simulink model "Collision_avoidance"  (R2025a)
settings: Solver=VariableStepAuto  StartTime=0.0  StopTime=30  RelTol=1e-3
InitFcn:
  | %% Simulation parameters and waypoint trajectory
  | % Initial drone positions.
  | init_0=[0;0;0];
  | d_s=4;
  | init_1=init_0+d_s*[-1.1;0.1;0];
  | init_2=init_0+d_s*[0.3;-1.5;0];
  | init_3=init_0+d_s*[0.2;1.8;0];
  | init_4=init_0+d_s*[1.6;0.4;0];
  | 
  | Threshold = 1000*ones(45,1);
  | for i=1:9:37
  |     Threshold(i:i+2)=10;
  | end
  | gain_2=1;
  | 
  | % Desired formation offsets.
  | init_f_0=[0;0;0];
  | d_f=1;
  | init_f_1=init_0+d_f*[0;-1;0];
  | init_f_2=init_0+d_f*[-1;0;0];
  | init_f_3=init_0+d_f*[1;0;0];
  | init_f_4=init_0+d_f*[0;1;0];
  | 
  | % Quadrotor mass and inertia.
  | mass = 1.2;
  | Ib   = diag([1.2416 1.2416 2*1.2416]);
  | 
  | % Time grid and waypoint trajectory.
  | Ts        = 0.001;
  | ttot      = 20;
  | tdead     = 10;
  | totalTime = ttot + tdead;
  | Nsamples  = 3000;
  | t_sample  = linspace(0, totalTime, Nsamples);
  | t=t_sample;
  | waypoints = [ ...
  |              0  0 0 0;
  |              0  0 0 0;
  |              0  0 0 0;
  |              0 0 0 0];
  | 
  | M    = size(waypoints,1);
  | t_wp = linspace(0, ttot, M);
  | 
  | p_d      = zeros(4, Nsamples);
  | dot_p_d  = zeros(4, Nsamples);
  | ddot_p_d = zeros(4, Nsamples);
  | 
  | idx_traj = t_sample <= ttot;
  | t_active = t_sample(idx_traj);
  | 
  | % Build position and yaw splines with zero endpoint velocities.
  | for dim = 1:4
  |     pp  = spline(t_wp, [0, waypoints(:,dim)&apos;, 0]);
  |     pp1 = fnder(pp,1);
  |     pp2 = fnder(pp,2);
  | 
  |     p_d(dim,    idx_traj) = ppval(pp,  t_active);
  |     dot_p_d(dim,idx_traj) = ppval(pp1, t_active);
  |     ddot_p_d(dim,idx_traj)= ppval(pp2, t_active);
  | end
  | 
  | % Hold the final waypoint after the maneuver.
  | last_wp_idx = M;
  | p_d(:, ~idx_traj)      = repmat(waypoints(last_wp_idx,:)&apos;, 1, sum(~idx_traj));
  | dot_p_d(:, ~idx_traj)  = 0;
  | ddot_p_d(:, ~idx_traj) = 0;
  | 
  | % Reference signals used by the Simulink blocks.
  | csi_d      = p_d(1:3,:);
  | psi_d      = p_d(4,:);
  | 
  | dot_csi_d  = dot_p_d(1:3,:);
  | ddot_csi_d = ddot_p_d(1:3,:);
  | dot_psi_d  = dot_p_d(4,:);
  | ddot_psi_d = ddot_p_d(4,:);
  | 
  | pos_0     = waypoints(1,1:3);
  | lin_vel_0 = [0 0 0];
  | w_bb_0    = [0 0 0];
undefined symbols (not defined in the file): A_diacenza, K
libraries: robotcorelib x5, uavutilslib x1
(part 1 of 2)
settings Model: Creator=fabioruggiero  LastModifiedBy=Giammo
settings ModelReferenceCC: EnableRefExpFcnMdlSchedulingChecks=on
settings RTWCC: GPUComputeCapability=3.5

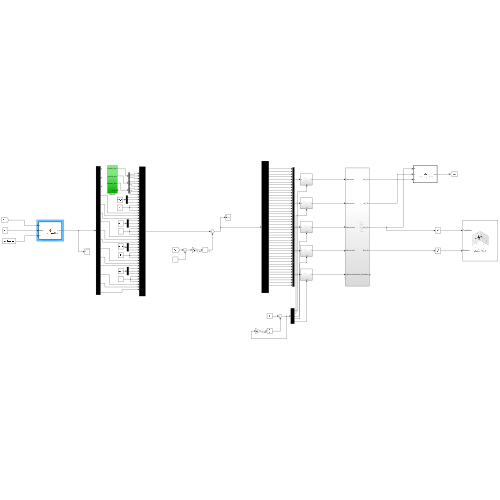
[thumbnail: Simulink's stored preview of the top-level diagram]
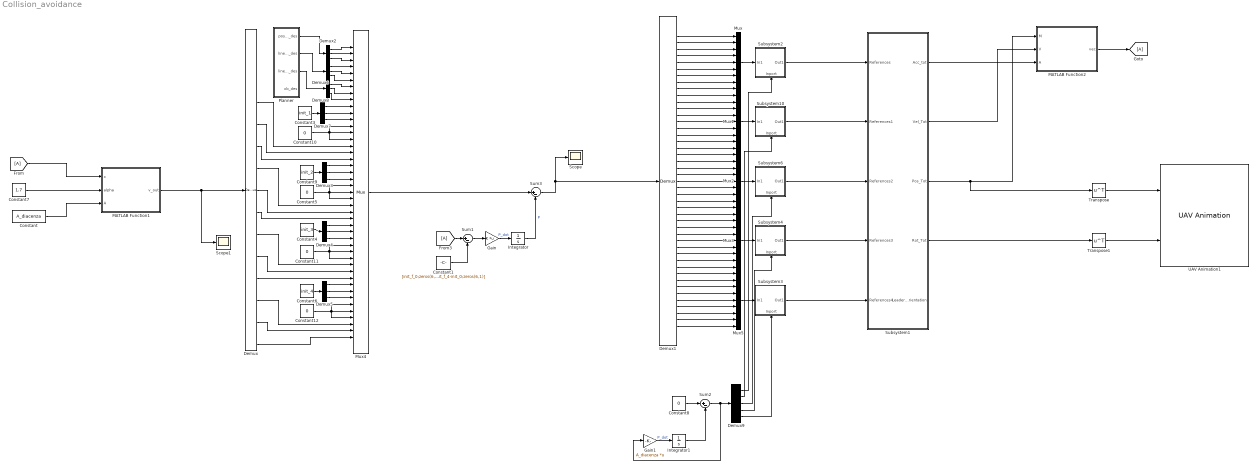
== system Collision_avoidance ==
  Constant : Constant  Value=A_diacenza
  Constant1 : Constant  Value=[init_f_0;zeros(6,1);init_f_1-init_0;zeros(6,1);init_f_2-init_0;zeros(6,1);init_f_3-init_0;zeros(6,1);init_f_4-init_0;zeros(6,1)]
  Constant{5,8,10..12} (5 alike) : Constant  Value=0
  Constant3 : Constant  Value=init_1
  Constant4 : Constant  Value=init_3
  Constant6 : Constant  Value=init_4
  Constant7 : Constant  Value=1.7
  Constant9 : Constant  Value=init_2
  Demux : Demux  Outputs=15
  Demux1 : Demux  Outputs=45
  Demux{2..8} (7 alike) : Demux  Outputs=3
  Demux9 : Demux  Outputs=5
  From : From
  From3 : From
  Gain : Gain  Gain=K  Multiplication=Matrix(K*u)
  Gain1 : Gain  Gain=A_diacenza  Multiplication=Matrix(K*u)
  Goto : Goto
  Integrator : Integrator
  Integrator1 : Integrator
  MATLAB Function1 : MATLAB Function  TreatAsAtomicUnit=on
  MATLAB Function2 : MATLAB Function  TreatAsAtomicUnit=on
  Mux{,1..3,5} (5 alike) : Mux  Inputs=9
  Mux4 : Mux  Inputs=45
  Planner : Subsystem
  Scope : Scope
      settings: ActiveDisplayYMinimum=-34.636381337350009  ActiveDisplayYMaximum=35.165535436651609  DataLoggingVariableName=ScopeData6
  Scope1 : Scope
      settings: ActiveDisplayYMinimum=-76.54569903346453  ActiveDisplayYMaximum=69.602196273492  DataLoggingVariableName=ScopeData7
  Subsystem1 : Subsystem
  Subsystem10 : Subsystem
      settings: PortSchema="{\"entries\":[{\"content\":{\"sides\":[{\"content\":{\"connectorIds\":[\"In1\"]},\"type\":\"ConnectorPlacement.EquallySpacedRectSide\",\"uuid\":\"6e5d8b99-8054-458f-abbe-7e3d6126420c\"},{\"content\":{\"connectorIds\":[\"Out1\"],\"side\":\"RIGHT\"},\"type\":\"ConnectorPlacement.EquallySpacedRectSide\",\"uuid\":\"d8af8c34-1227-4a19-bfdc-b42d943ed13c\"},{\"content\":{\"side\":\"TOP\"},\"type\":\"ConnectorPlacement.EquallySpacedRectSide\",\"uuid\":\"9c10b933-2873-4349-b535-f2af5c16ec70\"},{\"content\":{\"connectorIds\":[\"In2\"],\"side\":\"BOTTOM\"},\"type\":\"ConnectorPlacement.EquallySpacedRectSide\",\"uuid\":\"05be8d01-ed26-4f96-bcb1-0e501cb43bcc\"}]},\"type\":\"ConnectorPlacement.EquallySpacedConnector\",\"uuid\":\"f87e25de-488b-44c6-b2e5-9d22d609821c\"}],\"packageUris\":[\"http://schema.mathworks.com/mf0/Connector/R2020b\"],\"version\":\"1.0\"}"
  Subsystem2 : Subsystem
      settings: PortSchema="{\"entries\":[{\"content\":{\"sides\":[{\"content\":{\"connectorIds\":[\"In1\"]},\"type\":\"ConnectorPlacement.EquallySpacedRectSide\",\"uuid\":\"6e5d8b99-8054-458f-abbe-7e3d6126420c\"},{\"content\":{\"connectorIds\":[\"Out1\"],\"side\":\"RIGHT\"},\"type\":\"ConnectorPlacement.EquallySpacedRectSide\",\"uuid\":\"d8af8c34-1227-4a19-bfdc-b42d943ed13c\"},{\"content\":{\"side\":\"TOP\"},\"type\":\"ConnectorPlacement.EquallySpacedRectSide\",\"uuid\":\"9c10b933-2873-4349-b535-f2af5c16ec70\"},{\"content\":{\"connectorIds\":[\"In2\"],\"side\":\"BOTTOM\"},\"type\":\"ConnectorPlacement.EquallySpacedRectSide\",\"uuid\":\"05be8d01-ed26-4f96-bcb1-0e501cb43bcc\"}]},\"type\":\"ConnectorPlacement.EquallySpacedConnector\",\"uuid\":\"f87e25de-488b-44c6-b2e5-9d22d609821c\"}],\"packageUris\":[\"http://schema.mathworks.com/mf0/Connector/R2020b\"],\"version\":\"1.0\"}"
  Subsystem3 : Subsystem
      settings: PortSchema="{\"entries\":[{\"content\":{\"sides\":[{\"content\":{\"connectorIds\":[\"In1\"]},\"type\":\"ConnectorPlacement.EquallySpacedRectSide\",\"uuid\":\"6e5d8b99-8054-458f-abbe-7e3d6126420c\"},{\"content\":{\"connectorIds\":[\"Out1\"],\"side\":\"RIGHT\"},\"type\":\"ConnectorPlacement.EquallySpacedRectSide\",\"uuid\":\"d8af8c34-1227-4a19-bfdc-b42d943ed13c\"},{\"content\":{\"side\":\"TOP\"},\"type\":\"ConnectorPlacement.EquallySpacedRectSide\",\"uuid\":\"9c10b933-2873-4349-b535-f2af5c16ec70\"},{\"content\":{\"connectorIds\":[\"In2\"],\"side\":\"BOTTOM\"},\"type\":\"ConnectorPlacement.EquallySpacedRectSide\",\"uuid\":\"05be8d01-ed26-4f96-bcb1-0e501cb43bcc\"}]},\"type\":\"ConnectorPlacement.EquallySpacedConnector\",\"uuid\":\"f87e25de-488b-44c6-b2e5-9d22d609821c\"}],\"packageUris\":[\"http://schema.mathworks.com/mf0/Connector/R2020b\"],\"version\":\"1.0\"}"
  Subsystem4 : Subsystem
      settings: PortSchema="{\"entries\":[{\"content\":{\"sides\":[{\"content\":{\"connectorIds\":[\"In1\"]},\"type\":\"ConnectorPlacement.EquallySpacedRectSide\",\"uuid\":\"6e5d8b99-8054-458f-abbe-7e3d6126420c\"},{\"content\":{\"connectorIds\":[\"Out1\"],\"side\":\"RIGHT\"},\"type\":\"ConnectorPlacement.EquallySpacedRectSide\",\"uuid\":\"d8af8c34-1227-4a19-bfdc-b42d943ed13c\"},{\"content\":{\"side\":\"TOP\"},\"type\":\"ConnectorPlacement.EquallySpacedRectSide\",\"uuid\":\"9c10b933-2873-4349-b535-f2af5c16ec70\"},{\"content\":{\"connectorIds\":[\"In2\"],\"side\":\"BOTTOM\"},\"type\":\"ConnectorPlacement.EquallySpacedRectSide\",\"uuid\":\"05be8d01-ed26-4f96-bcb1-0e501cb43bcc\"}]},\"type\":\"ConnectorPlacement.EquallySpacedConnector\",\"uuid\":\"f87e25de-488b-44c6-b2e5-9d22d609821c\"}],\"packageUris\":[\"http://schema.mathworks.com/mf0/Connector/R2020b\"],\"version\":\"1.0\"}"
  Subsystem6 : Subsystem
      settings: PortSchema="{\"entries\":[{\"content\":{\"sides\":[{\"content\":{\"connectorIds\":[\"In1\"]},\"type\":\"ConnectorPlacement.EquallySpacedRectSide\",\"uuid\":\"6e5d8b99-8054-458f-abbe-7e3d6126420c\"},{\"content\":{\"connectorIds\":[\"Out1\"],\"side\":\"RIGHT\"},\"type\":\"ConnectorPlacement.EquallySpacedRectSide\",\"uuid\":\"d8af8c34-1227-4a19-bfdc-b42d943ed13c\"},{\"content\":{\"side\":\"TOP\"},\"type\":\"ConnectorPlacement.EquallySpacedRectSide\",\"uuid\":\"9c10b933-2873-4349-b535-f2af5c16ec70\"},{\"content\":{\"connectorIds\":[\"In2\"],\"side\":\"BOTTOM\"},\"type\":\"ConnectorPlacement.EquallySpacedRectSide\",\"uuid\":\"05be8d01-ed26-4f96-bcb1-0e501cb43bcc\"}]},\"type\":\"ConnectorPlacement.EquallySpacedConnector\",\"uuid\":\"f87e25de-488b-44c6-b2e5-9d22d609821c\"}],\"packageUris\":[\"http://schema.mathworks.com/mf0/Connector/R2020b\"],\"version\":\"1.0\"}"
  Sum1 : Sum  Inputs=|+-
  Sum2 : Sum  Inputs=|+-
  Sum3 : Sum  Inputs=|+-
  Transpose : Math  Operator=transpose
  Transpose1 : Math  Operator=transpose
  UAV Animation1 : uavutilslib/UAV Animation  NumUAV=5  DynamicUAVConfig=off  UAVType=Multirotor  UAVSize=1  UAVColor=[1 0 0]  UAVTrajectoryAlpha=1  InertialZDirection=Down  RotationFormat=Quaternion  DrawMarkers=off  SampleTime=0.01
  wires:
  Demux9/5 -> Subsystem3/2(Inport)
  Transpose1/1 -> UAV Animation1/2
  Transpose/1 -> UAV Animation1/1
  Sum2/1 -> Demux9/1, Gain1/1
  Gain1/1 -> Integrator1/1  "P_dot"
  Integrator1/1 -> Sum2/2
  Mux3/1 -> Subsystem4/1(In1)
  Mux/1 -> Subsystem2/1(In1)
  Subsystem2/1(Out1) -> Subsystem1/1(References)
  Demux9/2 -> Subsystem10/2(Inport)
  Subsystem3/1(Out1) -> Subsystem1/5(References4)
  Mux5/1 -> Subsystem3/1(In1)
  Subsystem6/1(Out1) -> Subsystem1/3(References2)
  Mux2/1 -> Subsystem6/1(In1)
  Subsystem1/2(Vel_Tot) -> MATLAB Function2/2(V)
  Demux1/1 -> Mux/1
  Demux1/15 -> Mux1/6
  Demux9/1 -> Subsystem2/2(Inport)
  Demux1/23 -> Mux2/5
  Demux1/12 -> Mux1/3
  Demux1/4 -> Mux/4
  Demux1/31 -> Mux3/4
  Demux1/41 -> Mux5/5
  Demux1/19 -> Mux2/1
  Demux1/26 -> Mux2/8
  Demux1/29 -> Mux3/2
  Demux1/34 -> Mux3/7
  Demux1/39 -> Mux5/3
  Demux1/20 -> Mux2/2
  Demux1/38 -> Mux5/2
  Demux1/43 -> Mux5/7
  Demux1/42 -> Mux5/6
  Demux1/30 -> Mux3/3
  Demux1/36 -> Mux3/9
  From/1 -> MATLAB Function1/1(x)
  Demux1/27 -> Mux2/9
  Demux9/4 -> Subsystem4/2(Inport)
  Subsystem1/1(Acc_tot) -> MATLAB Function2/3(A)
  Demux1/22 -> Mux2/4
  Subsystem1/3(Pos_Tot) -> Transpose/1, MATLAB Function2/1(M)
  Demux1/32 -> Mux3/5
  Demux1/14 -> Mux1/5
  Demux1/13 -> Mux1/4
  Demux1/21 -> Mux2/3
  Demux1/33 -> Mux3/6
  Subsystem1/4(Rot_Tot) -> Transpose1/1
  Demux1/9 -> Mux/9
  Mux1/1 -> Subsystem10/1(In1)
  Demux1/40 -> Mux5/4
  Demux1/3 -> Mux/3
  Demux1/6 -> Mux/6
  Demux1/25 -> Mux2/7
  Demux1/8 -> Mux/8
  Demux1/28 -> Mux3/1
  Demux1/10 -> Mux1/1
  Demux1/7 -> Mux/7
  Demux1/37 -> Mux5/1
  Demux1/11 -> Mux1/2
  Demux1/45 -> Mux5/9
  Demux1/17 -> Mux1/8
  Demux1/35 -> Mux3/8
  Demux1/5 -> Mux/5
  Demux1/44 -> Mux5/8
  Constant11/1 -> Mux4/31, Mux4/33, Mux4/32
  Planner/3(linear_acceleration_des) -> Demux8/1
  Demux1/18 -> Mux1/9
  Demux/9 -> Mux4/27
  Demux1/16 -> Mux1/7
  Demux1/2 -> Mux/2
  Constant7/1 -> MATLAB Function1/2(alpha)
  Constant12/1 -> Mux4/40, Mux4/41, Mux4/42
  Constant10/1 -> Mux4/13, Mux4/15, Mux4/14
  Demux4/3 -> Mux4/30
  Mux4/1 -> Sum3/1
  Demux3/2 -> Mux4/20
  Demux2/2 -> Mux4/2
  Constant3/1 -> Demux7/1
  Demux5/2 -> Mux4/38
  Demux8/2 -> Mux4/8
  Constant8/1 -> Sum2/1
  Demux2/1 -> Mux4/1
  Demux7/2 -> Mux4/11
  Demux8/1 -> Mux4/7
  Demux2/3 -> Mux4/3
  Constant5/1 -> Mux4/22, Mux4/24, Mux4/23
  Demux/6 -> Mux4/18
  MATLAB Function1/1(v_out) -> Scope1/1, Demux/1
  Demux3/3 -> Mux4/21
  Demux6/1 -> Mux4/4
  Demux/5 -> Mux4/17
  Demux8/3 -> Mux4/9
  Demux/12 -> Mux4/36
  Constant4/1 -> Demux4/1
  Demux6/2 -> Mux4/5
  Demux/7 -> Mux4/25
  Demux/14 -> Mux4/44
  Constant6/1 -> Demux5/1
  Constant9/1 -> Demux3/1
  Demux5/3 -> Mux4/39
  Demux/8 -> Mux4/26
  Demux7/1 -> Mux4/10
  Demux7/3 -> Mux4/12
  Planner/2(linear_velocity_des) -> Demux6/1
  Constant/1 -> MATLAB Function1/3(A)
  Sum3/1 -> Demux1/1, Scope/1
  Subsystem4/1(Out1) -> Subsystem1/4(References3)
  Demux3/1 -> Mux4/19
  Demux4/1 -> Mux4/28
  Demux4/2 -> Mux4/29
  Demux/10 -> Mux4/34
  Demux6/3 -> Mux4/6
  Demux/4 -> Mux4/16
  Planner/1(position_des) -> Demux2/1
  Demux5/1 -> Mux4/37
  Demux/11 -> Mux4/35
  Demux/15 -> Mux4/45
  Demux9/3 -> Subsystem6/2(Inport)
  Demux1/24 -> Mux2/6
  Subsystem10/1(Out1) -> Subsystem1/2(References1)
  Demux/13 -> Mux4/43
  MATLAB Function2/1(vec) -> Goto/1
  Constant1/1 -> Sum1/2
  From3/1 -> Sum1/1
  Sum1/1 -> Gain/1
  Gain/1 -> Integrator/1  "P_dot"
  Integrator/1 -> Sum3/2  "P"

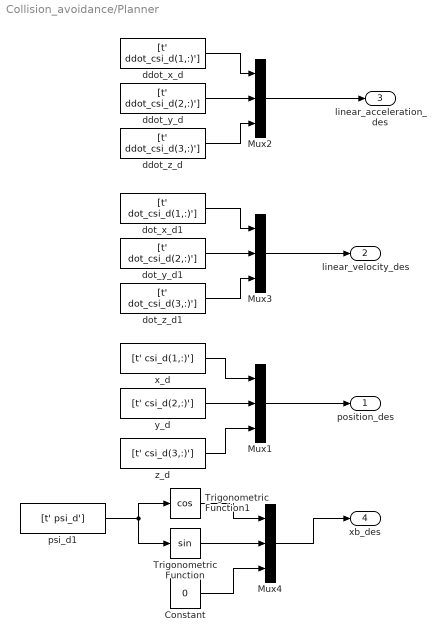
== system Collision_avoidance/Planner ==
  Constant : Constant  Value=0
  Mux{1..4} (4 alike) : Mux  Inputs=3
  Trigonometric Function : Trigonometry
  Trigonometric Function1 : Trigonometry  Operator=cos
  ddot_x_d : FromWorkspace  VariableName=[t' ddot_csi_d(1,:)']  SampleTime=Ts
  ddot_y_d : FromWorkspace  VariableName=[t' ddot_csi_d(2,:)']  SampleTime=Ts
  ddot_z_d : FromWorkspace  VariableName=[t' ddot_csi_d(3,:)']  SampleTime=Ts
  dot_x_d1 : FromWorkspace  VariableName=[t' dot_csi_d(1,:)']  SampleTime=Ts
  dot_y_d1 : FromWorkspace  VariableName=[t' dot_csi_d(2,:)']  SampleTime=Ts
  dot_z_d1 : FromWorkspace  VariableName=[t' dot_csi_d(3,:)']  SampleTime=Ts
  psi_d1 : FromWorkspace  VariableName=[t' psi_d']  SampleTime=Ts
  x_d : FromWorkspace  VariableName=[t' csi_d(1,:)']  SampleTime=Ts
  y_d : FromWorkspace  VariableName=[t' csi_d(2,:)']  SampleTime=Ts
  z_d : FromWorkspace  VariableName=[t' csi_d(3,:)']  SampleTime=Ts
  position_des : Outport
  linear_velocity_des : Outport  Port=2
  linear_acceleration_des : Outport  Port=3
  xb_des : Outport  Port=4
  wires:
  y_d/1 -> Mux1/2
  z_d/1 -> Mux1/3
  x_d/1 -> Mux1/1
  ddot_y_d/1 -> Mux2/2
  ddot_z_d/1 -> Mux2/3
  ddot_x_d/1 -> Mux2/1
  Mux2/1 -> linear_acceleration_des/1
  Mux1/1 -> position_des/1
  dot_y_d1/1 -> Mux3/2
  dot_z_d1/1 -> Mux3/3
  dot_x_d1/1 -> Mux3/1
  Mux3/1 -> linear_velocity_des/1
  Mux4/1 -> xb_des/1
  Trigonometric Function/1 -> Mux4/2
  psi_d1/1 -> Trigonometric Function/1, Trigonometric Function1/1
  Trigonometric Function1/1 -> Mux4/1
  Constant/1 -> Mux4/3

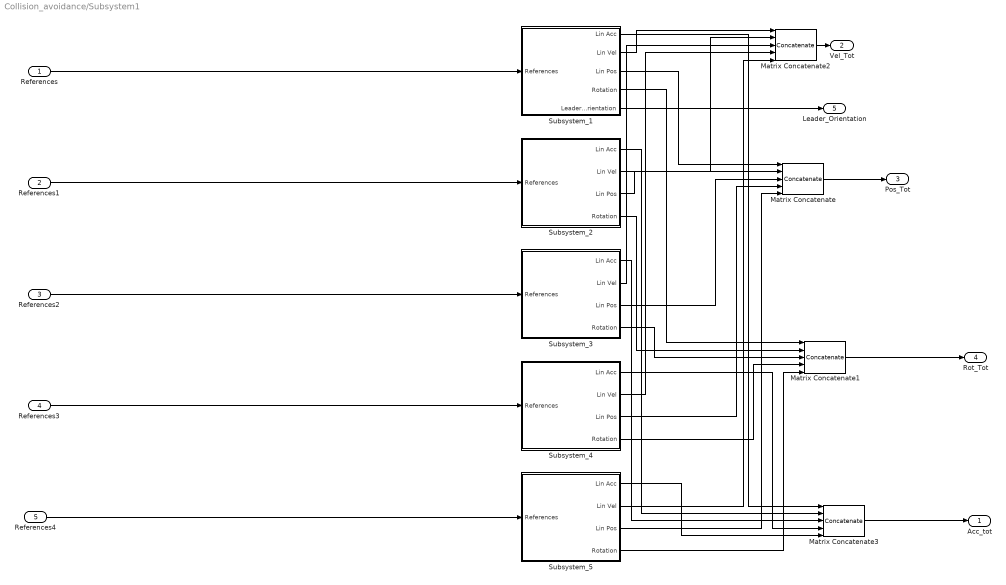
== system Collision_avoidance/Subsystem1 ==
  References : Inport
  References1 : Inport  Port=2
  References2 : Inport  Port=3
  References3 : Inport  Port=4
  References4 : Inport  Port=5
  Matrix Concatenate{,1..3} (4 alike) : Concatenate  NumInputs=5  Mode=Multidimensional array  ConcatenateDimension=2
  Subsystem_1 : Subsystem
  Subsystem_2 : Subsystem
  Subsystem_3 : Subsystem
  Subsystem_4 : Subsystem
  Subsystem_5 : Subsystem
  Acc_tot : Outport
  Vel_Tot : Outport  Port=2
  Pos_Tot : Outport  Port=3
  Rot_Tot : Outport  Port=4
  Leader_Orientation : Outport  Port=5
  wires:
  Matrix Concatenate3/1 -> Acc_tot/1
  Subsystem_1/1(Lin Acc) -> Matrix Concatenate3/1
  Subsystem_3/1(Lin Acc) -> Matrix Concatenate3/3
  Subsystem_5/1(Lin Acc) -> Matrix Concatenate3/5
  References1/1 -> Subsystem_2/1(References)
  Matrix Concatenate1/1 -> Rot_Tot/1
  References2/1 -> Subsystem_3/1(References)
  References3/1 -> Subsystem_4/1(References)
  References/1 -> Subsystem_1/1(References)
  Matrix Concatenate/1 -> Pos_Tot/1
  References4/1 -> Subsystem_5/1(References)
  Subsystem_5/2(Lin Vel) -> Matrix Concatenate2/5
  Subsystem_4/2(Lin Vel) -> Matrix Concatenate2/4
  Subsystem_4/1(Lin Acc) -> Matrix Concatenate3/4
  Subsystem_1/2(Lin Vel) -> Matrix Concatenate2/1
  Matrix Concatenate2/1 -> Vel_Tot/1
  Subsystem_3/3(Lin Pos) -> Matrix Concatenate/3
  Subsystem_2/1(Lin Acc) -> Matrix Concatenate3/2
  Subsystem_1/3(Lin Pos) -> Matrix Concatenate/1
  Subsystem_3/4(Rotation) -> Matrix Concatenate1/3
  Subsystem_5/3(Lin Pos) -> Matrix Concatenate/5
  Subsystem_2/4(Rotation) -> Matrix Concatenate1/2
  Subsystem_1/4(Rotation) -> Matrix Concatenate1/1
  Subsystem_4/4(Rotation) -> Matrix Concatenate1/4
  Subsystem_3/2(Lin Vel) -> Matrix Concatenate2/3
  Subsystem_2/3(Lin Pos) -> Matrix Concatenate/2
  Subsystem_5/4(Rotation) -> Matrix Concatenate1/5
  Subsystem_2/2(Lin Vel) -> Matrix Concatenate2/2
  Subsystem_4/3(Lin Pos) -> Matrix Concatenate/4
  Subsystem_1/5(Leader_Orientation) -> Leader_Orientation/1

== system Collision_avoidance/Subsystem10 ==
  In1 : Inport
  Inport : Inport  Port=2
  Constant1 : Constant  Value=[0;0;0]
  Demux : Demux  Outputs=9
  Demux1 : Demux  Outputs=3
  Mux : Mux  Inputs=3
  Mux2 : Mux  Inputs=10
  Sum : Sum  Inputs=++|
  Out1 : Outport
  wires:
  Mux2/1 -> Out1/1
  In1/1 -> Demux/1
  Demux/4 -> Mux2/4
  Demux/5 -> Mux2/5
  Demux/6 -> Mux2/6
  Demux/7 -> Mux2/7
  Demux/8 -> Mux2/8
  Demux/9 -> Mux2/9
  Demux/1 -> Mux/1
  Demux/2 -> Mux/2
  Demux/3 -> Mux/3
  Mux/1 -> Sum/2
  Constant1/1 -> Sum/1
  Sum/1 -> Demux1/1
  Demux1/1 -> Mux2/1
  Demux1/2 -> Mux2/2
  Demux1/3 -> Mux2/3
  Inport/1 -> Mux2/10

== system Collision_avoidance/Subsystem2 ==
  In1 : Inport
  Inport : Inport  Port=2
  Constant1 : Constant  Value=[0;0;0]
  Demux : Demux  Outputs=9
  Demux1 : Demux  Outputs=3
  Mux : Mux  Inputs=3
  Mux2 : Mux  Inputs=10
  Sum : Sum  Inputs=++|
  Out1 : Outport
  wires:
  Mux2/1 -> Out1/1
  In1/1 -> Demux/1
  Demux/4 -> Mux2/4
  Demux/5 -> Mux2/5
  Demux/6 -> Mux2/6
  Demux/7 -> Mux2/7
  Demux/8 -> Mux2/8
  Demux/9 -> Mux2/9
  Demux/1 -> Mux/1
  Demux/2 -> Mux/2
  Demux/3 -> Mux/3
  Mux/1 -> Sum/2
  Constant1/1 -> Sum/1
  Sum/1 -> Demux1/1
  Demux1/1 -> Mux2/1
  Demux1/2 -> Mux2/2
  Demux1/3 -> Mux2/3
  Inport/1 -> Mux2/10

== system Collision_avoidance/Subsystem3 ==
  In1 : Inport
  Inport : Inport  Port=2
  Constant1 : Constant  Value=[0;0;0]
  Demux : Demux  Outputs=9
  Demux1 : Demux  Outputs=3
  Mux : Mux  Inputs=3
  Mux2 : Mux  Inputs=10
  Sum : Sum  Inputs=++|
  Out1 : Outport
  wires:
  Mux2/1 -> Out1/1
  In1/1 -> Demux/1
  Demux/4 -> Mux2/4
  Demux/5 -> Mux2/5
  Demux/6 -> Mux2/6
  Demux/7 -> Mux2/7
  Demux/8 -> Mux2/8
  Demux/9 -> Mux2/9
  Demux/1 -> Mux/1
  Demux/2 -> Mux/2
  Demux/3 -> Mux/3
  Mux/1 -> Sum/2
  Constant1/1 -> Sum/1
  Sum/1 -> Demux1/1
  Demux1/1 -> Mux2/1
  Demux1/2 -> Mux2/2
  Demux1/3 -> Mux2/3
  Inport/1 -> Mux2/10

== system Collision_avoidance/Subsystem4 ==
  In1 : Inport
  Inport : Inport  Port=2
  Constant1 : Constant  Value=[0;0;0]
  Demux : Demux  Outputs=9
  Demux1 : Demux  Outputs=3
  Mux : Mux  Inputs=3
  Mux2 : Mux  Inputs=10
  Sum : Sum  Inputs=++|
  Out1 : Outport
  wires:
  Mux2/1 -> Out1/1
  In1/1 -> Demux/1
  Demux/4 -> Mux2/4
  Demux/5 -> Mux2/5
  Demux/6 -> Mux2/6
  Demux/7 -> Mux2/7
  Demux/8 -> Mux2/8
  Demux/9 -> Mux2/9
  Demux/1 -> Mux/1
  Demux/2 -> Mux/2
  Demux/3 -> Mux/3
  Mux/1 -> Sum/2
  Constant1/1 -> Sum/1
  Sum/1 -> Demux1/1
  Demux1/1 -> Mux2/1
  Demux1/2 -> Mux2/2
  Demux1/3 -> Mux2/3
  Inport/1 -> Mux2/10

== system Collision_avoidance/Subsystem6 ==
  In1 : Inport
  Inport : Inport  Port=2
  Constant1 : Constant  Value=[0;0;0]
  Demux : Demux  Outputs=9
  Demux1 : Demux  Outputs=3
  Mux : Mux  Inputs=3
  Mux2 : Mux  Inputs=10
  Sum : Sum  Inputs=++|
  Out1 : Outport
  wires:
  Mux2/1 -> Out1/1
  In1/1 -> Demux/1
  Demux/4 -> Mux2/4
  Demux/5 -> Mux2/5
  Demux/6 -> Mux2/6
  Demux/7 -> Mux2/7
  Demux/8 -> Mux2/8
  Demux/9 -> Mux2/9
  Demux/1 -> Mux/1
  Demux/2 -> Mux/2
  Demux/3 -> Mux/3
  Mux/1 -> Sum/2
  Constant1/1 -> Sum/1
  Sum/1 -> Demux1/1
  Demux1/1 -> Mux2/1
  Demux1/2 -> Mux2/2
  Demux1/3 -> Mux2/3
  Inport/1 -> Mux2/10

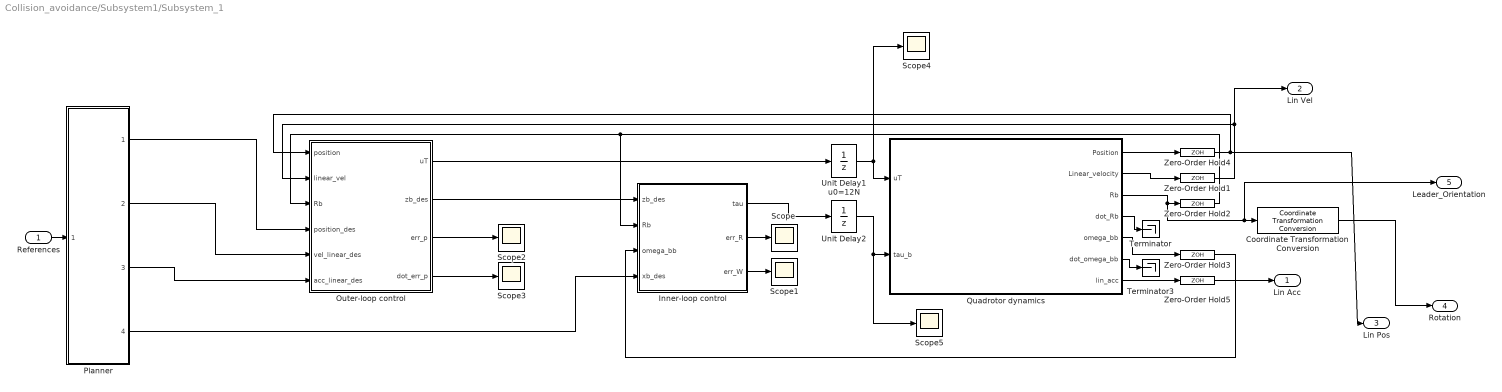
== system Collision_avoidance/Subsystem1/Subsystem_1 ==
  References : Inport
  Coordinate Transformation Conversion : robotcorelib/Coordinate Transformation Conversion  InputRepresentation=Rotation Matrix  InputEulerSequence=ZYX  ShowTrVecInputPort=on  OutputRepresentation=Quaternion  OutputEulerSequence=ZYX  ShowTrVecOutputPort=on  SimulateUsing=Interpreted execution
  Inner-loop control : Subsystem
  Outer-loop control : MATLAB Function  TreatAsAtomicUnit=on
  Planner : Subsystem
  Quadrotor dynamics : Subsystem
  Scope{,1..5} (6 alike) : Scope
      Scope settings: ActiveDisplayYMinimum=-1.2E-5  ActiveDisplayYMaximum=1.2E-5
      Scope1 settings: ActiveDisplayYMinimum=-1.2E-5  ActiveDisplayYMaximum=1.2E-5
      Scope2 settings: ActiveDisplayYMinimum=-3.9E-5  ActiveDisplayYMaximum=1.1E-5  DataLoggingVariableName=ScopeData2
      Scope3 settings: ActiveDisplayYMinimum=-0.00022  ActiveDisplayYMaximum=0.00011  DataLoggingVariableName=ScopeData3
      Scope4 settings: ActiveDisplayYMinimum=11.66748  ActiveDisplayYMaximum=12.03695  DataLoggingVariableName=ScopeData4
      Scope5 settings: ActiveDisplayYMinimum=-0.02035  ActiveDisplayYMaximum=0.02036  DataLoggingVariableName=ScopeData5
  Terminator : Terminator
  Terminator3 : Terminator
  Unit Delay1 u0=12N : UnitDelay  InitialCondition=12  SampleTime=Ts
  Unit Delay2 : UnitDelay  InitialCondition=[0 0 0]  SampleTime=Ts
  Zero-Order Hold{1..5} (5 alike) : ZeroOrderHold  SampleTime=Ts
  Lin Acc : Outport
  Lin Vel : Outport  Port=2
  Lin Pos : Outport  Port=3
  Rotation : Outport  Port=4
  Leader_Orientation : Outport  Port=5
  wires:
  Zero-Order Hold5/1 -> Lin Acc/1
  Quadrotor dynamics/7(lin_acc) -> Zero-Order Hold5/1
  Planner/1(position_des) -> Outer-loop control/4(position_des)
  Quadrotor dynamics/1(Position) -> Zero-Order Hold4/1
  Quadrotor dynamics/3(Rb) -> Zero-Order Hold2/1, Leader_Orientation/1, Coordinate Transformation Conversion/1
  Quadrotor dynamics/4(dot_Rb) -> Terminator/1
  Planner/4(xb_des) -> Inner-loop control/4(xb_des)
  Inner-loop control/1(tau) -> Unit Delay2/1
  Planner/2(linear_velocity_des) -> Outer-loop control/5(vel_linear_des)
  Quadrotor dynamics/2(Linear_velocity) -> Zero-Order Hold1/1
  Quadrotor dynamics/6(dot_omega_bb) -> Terminator3/1
  Outer-loop control/3(err_p) -> Scope2/1
  Coordinate Transformation Conversion/1 -> Rotation/1
  Quadrotor dynamics/5(omega_bb) -> Zero-Order Hold3/1
  Zero-Order Hold2/1 -> Inner-loop control/2(Rb), Outer-loop control/3(Rb)
  References/1 -> Planner/1(References)
  Planner/3(linear_acceleration_des) -> Outer-loop control/6(acc_linear_des)
  Inner-loop control/3(err_W) -> Scope1/1
  Outer-loop control/2(zb_des) -> Inner-loop control/1(zb_des)
  Inner-loop control/2(err_R) -> Scope/1
  Outer-loop control/1(uT) -> Unit Delay1 u0=12N/1
  Unit Delay2/1 -> Quadrotor dynamics/2(tau_b), Scope5/1
  Zero-Order Hold3/1 -> Inner-loop control/3(omega_bb)
  Unit Delay1 u0=12N/1 -> Scope4/1, Quadrotor dynamics/1(uT)
  Outer-loop control/4(dot_err_p) -> Scope3/1
  Zero-Order Hold1/1 -> Outer-loop control/2(linear_vel), Lin Vel/1
  Zero-Order Hold4/1 -> Outer-loop control/1(position), Lin Pos/1

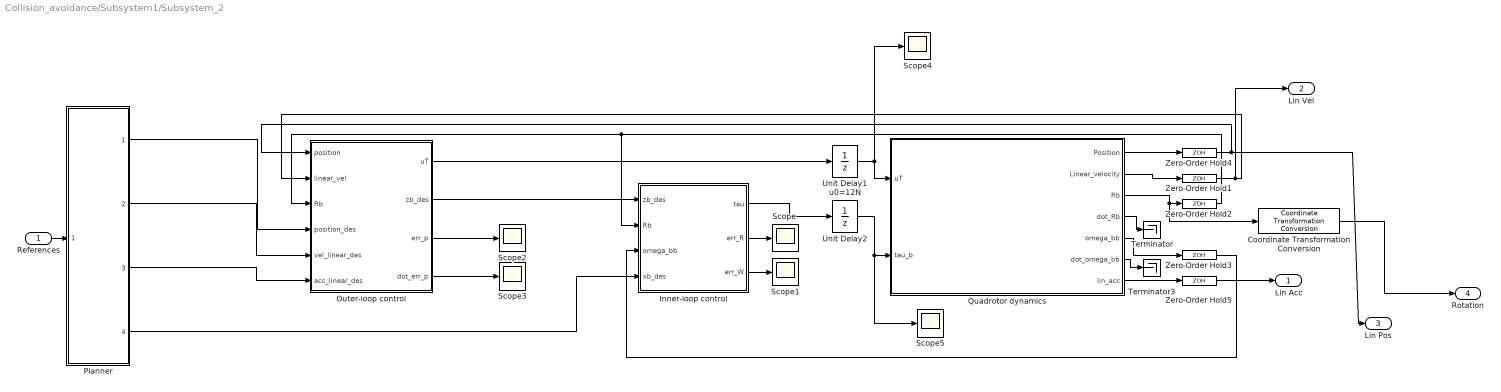
== system Collision_avoidance/Subsystem1/Subsystem_2 ==
  References : Inport
  Coordinate Transformation Conversion : robotcorelib/Coordinate Transformation Conversion  InputRepresentation=Rotation Matrix  InputEulerSequence=ZYX  ShowTrVecInputPort=on  OutputRepresentation=Quaternion  OutputEulerSequence=ZYX  ShowTrVecOutputPort=on  SimulateUsing=Interpreted execution
  Inner-loop control : Subsystem
  Outer-loop control : MATLAB Function  TreatAsAtomicUnit=on
  Planner : Subsystem
  Quadrotor dynamics : Subsystem
  Scope{,1..5} (6 alike) : Scope
      Scope settings: ActiveDisplayYMinimum=-1.2E-5  ActiveDisplayYMaximum=1.2E-5
      Scope1 settings: ActiveDisplayYMinimum=-1.2E-5  ActiveDisplayYMaximum=1.2E-5
      Scope2 settings: ActiveDisplayYMinimum=-3.9E-5  ActiveDisplayYMaximum=1.1E-5  DataLoggingVariableName=ScopeData2
      Scope3 settings: ActiveDisplayYMinimum=-0.00022  ActiveDisplayYMaximum=0.00011  DataLoggingVariableName=ScopeData3
      Scope4 settings: ActiveDisplayYMinimum=11.66748  ActiveDisplayYMaximum=12.03695  DataLoggingVariableName=ScopeData4
      Scope5 settings: ActiveDisplayYMinimum=-0.02035  ActiveDisplayYMaximum=0.02036  DataLoggingVariableName=ScopeData5
  Terminator : Terminator
  Terminator3 : Terminator
  Unit Delay1 u0=12N : UnitDelay  InitialCondition=12  SampleTime=Ts
  Unit Delay2 : UnitDelay  InitialCondition=[0 0 0]  SampleTime=Ts
  Zero-Order Hold{1..5} (5 alike) : ZeroOrderHold  SampleTime=Ts
  Lin Acc : Outport
  Lin Vel : Outport  Port=2
  Lin Pos : Outport  Port=3
  Rotation : Outport  Port=4
  wires:
  Zero-Order Hold5/1 -> Lin Acc/1
  Quadrotor dynamics/7(lin_acc) -> Zero-Order Hold5/1
  Planner/1(position_des) -> Outer-loop control/4(position_des)
  Quadrotor dynamics/1(Position) -> Zero-Order Hold4/1
  Quadrotor dynamics/3(Rb) -> Zero-Order Hold2/1, Coordinate Transformation Conversion/1
  Quadrotor dynamics/4(dot_Rb) -> Terminator/1
  Planner/4(xb_des) -> Inner-loop control/4(xb_des)
  Inner-loop control/1(tau) -> Unit Delay2/1
  Planner/2(linear_velocity_des) -> Outer-loop control/5(vel_linear_des)
  Quadrotor dynamics/2(Linear_velocity) -> Zero-Order Hold1/1
  Quadrotor dynamics/6(dot_omega_bb) -> Terminator3/1
  Outer-loop control/3(err_p) -> Scope2/1
  Coordinate Transformation Conversion/1 -> Rotation/1
  Quadrotor dynamics/5(omega_bb) -> Zero-Order Hold3/1
  Zero-Order Hold2/1 -> Inner-loop control/2(Rb), Outer-loop control/3(Rb)
  References/1 -> Planner/1(References)
  Planner/3(linear_acceleration_des) -> Outer-loop control/6(acc_linear_des)
  Inner-loop control/3(err_W) -> Scope1/1
  Outer-loop control/2(zb_des) -> Inner-loop control/1(zb_des)
  Inner-loop control/2(err_R) -> Scope/1
  Outer-loop control/1(uT) -> Unit Delay1 u0=12N/1
  Unit Delay2/1 -> Quadrotor dynamics/2(tau_b), Scope5/1
  Zero-Order Hold3/1 -> Inner-loop control/3(omega_bb)
  Unit Delay1 u0=12N/1 -> Scope4/1, Quadrotor dynamics/1(uT)
  Outer-loop control/4(dot_err_p) -> Scope3/1
  Zero-Order Hold1/1 -> Outer-loop control/2(linear_vel), Lin Vel/1
  Zero-Order Hold4/1 -> Outer-loop control/1(position), Lin Pos/1

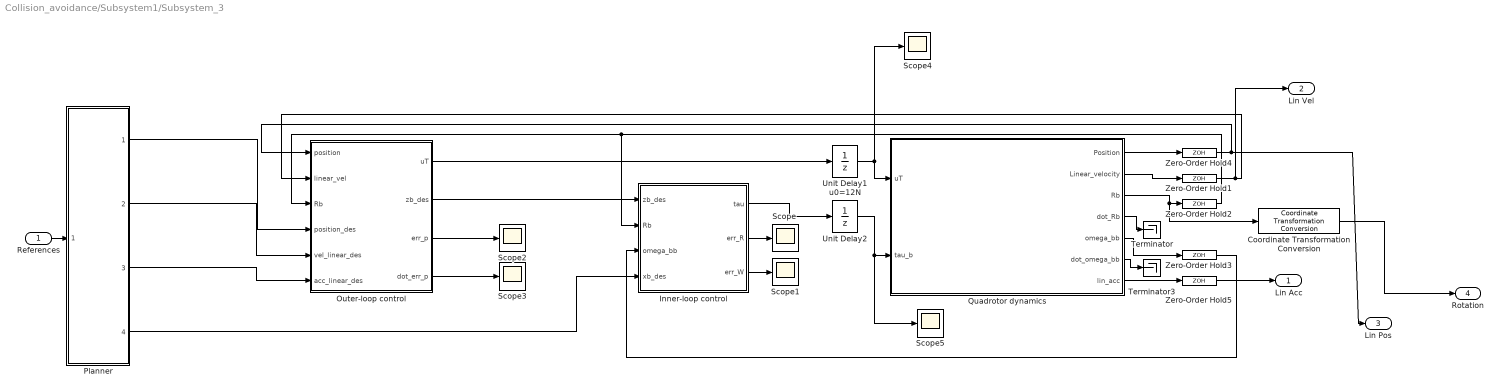
== system Collision_avoidance/Subsystem1/Subsystem_3 ==
  References : Inport
  Coordinate Transformation Conversion : robotcorelib/Coordinate Transformation Conversion  InputRepresentation=Rotation Matrix  InputEulerSequence=ZYX  ShowTrVecInputPort=on  OutputRepresentation=Quaternion  OutputEulerSequence=ZYX  ShowTrVecOutputPort=on  SimulateUsing=Interpreted execution
  Inner-loop control : Subsystem
  Outer-loop control : MATLAB Function  TreatAsAtomicUnit=on
  Planner : Subsystem
  Quadrotor dynamics : Subsystem
  Scope{,1..5} (6 alike) : Scope
      Scope settings: ActiveDisplayYMinimum=-1.2E-5  ActiveDisplayYMaximum=1.2E-5
      Scope1 settings: ActiveDisplayYMinimum=-1.2E-5  ActiveDisplayYMaximum=1.2E-5
      Scope2 settings: ActiveDisplayYMinimum=-3.9E-5  ActiveDisplayYMaximum=1.1E-5  DataLoggingVariableName=ScopeData2
      Scope3 settings: ActiveDisplayYMinimum=-0.00022  ActiveDisplayYMaximum=0.00011  DataLoggingVariableName=ScopeData3
      Scope4 settings: ActiveDisplayYMinimum=11.66748  ActiveDisplayYMaximum=12.03695  DataLoggingVariableName=ScopeData4
      Scope5 settings: ActiveDisplayYMinimum=-0.02035  ActiveDisplayYMaximum=0.02036  DataLoggingVariableName=ScopeData5
  Terminator : Terminator
  Terminator3 : Terminator
  Unit Delay1 u0=12N : UnitDelay  InitialCondition=12  SampleTime=Ts
  Unit Delay2 : UnitDelay  InitialCondition=[0 0 0]  SampleTime=Ts
  Zero-Order Hold{1..5} (5 alike) : ZeroOrderHold  SampleTime=Ts
  Lin Acc : Outport
  Lin Vel : Outport  Port=2
  Lin Pos : Outport  Port=3
  Rotation : Outport  Port=4
  wires:
  Zero-Order Hold5/1 -> Lin Acc/1
  Quadrotor dynamics/7(lin_acc) -> Zero-Order Hold5/1
  Planner/1(position_des) -> Outer-loop control/4(position_des)
  Quadrotor dynamics/1(Position) -> Zero-Order Hold4/1
  Quadrotor dynamics/3(Rb) -> Zero-Order Hold2/1, Coordinate Transformation Conversion/1
  Quadrotor dynamics/4(dot_Rb) -> Terminator/1
  Planner/4(xb_des) -> Inner-loop control/4(xb_des)
  Inner-loop control/1(tau) -> Unit Delay2/1
  Planner/2(linear_velocity_des) -> Outer-loop control/5(vel_linear_des)
  Quadrotor dynamics/2(Linear_velocity) -> Zero-Order Hold1/1
  Quadrotor dynamics/6(dot_omega_bb) -> Terminator3/1
  Outer-loop control/3(err_p) -> Scope2/1
  Coordinate Transformation Conversion/1 -> Rotation/1
  Quadrotor dynamics/5(omega_bb) -> Zero-Order Hold3/1
  Zero-Order Hold2/1 -> Inner-loop control/2(Rb), Outer-loop control/3(Rb)
  References/1 -> Planner/1(References)
  Planner/3(linear_acceleration_des) -> Outer-loop control/6(acc_linear_des)
  Inner-loop control/3(err_W) -> Scope1/1
  Outer-loop control/2(zb_des) -> Inner-loop control/1(zb_des)
  Inner-loop control/2(err_R) -> Scope/1
  Outer-loop control/1(uT) -> Unit Delay1 u0=12N/1
  Unit Delay2/1 -> Quadrotor dynamics/2(tau_b), Scope5/1
  Zero-Order Hold3/1 -> Inner-loop control/3(omega_bb)
  Unit Delay1 u0=12N/1 -> Scope4/1, Quadrotor dynamics/1(uT)
  Outer-loop control/4(dot_err_p) -> Scope3/1
  Zero-Order Hold1/1 -> Outer-loop control/2(linear_vel), Lin Vel/1
  Zero-Order Hold4/1 -> Outer-loop control/1(position), Lin Pos/1

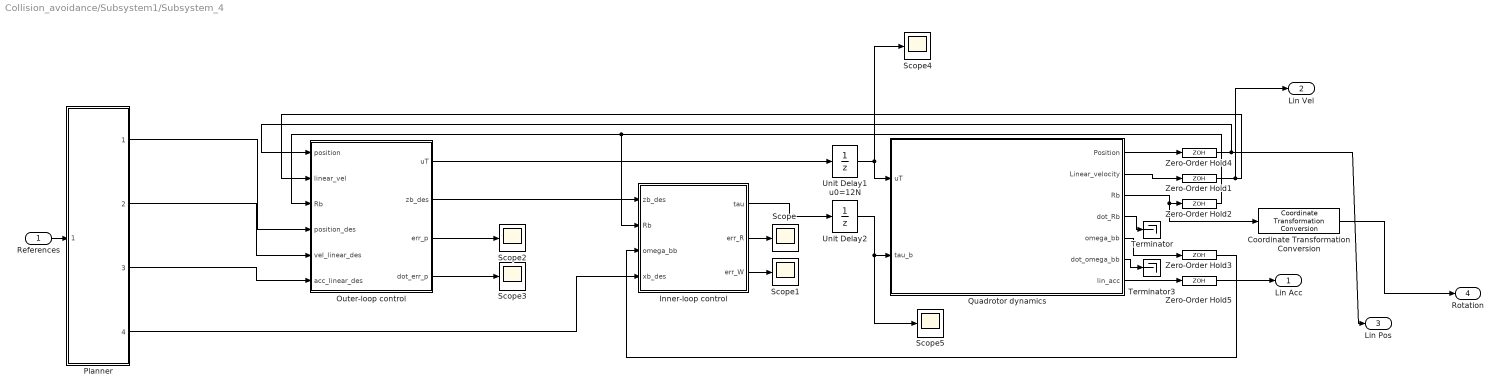
== system Collision_avoidance/Subsystem1/Subsystem_4 ==
  References : Inport
  Coordinate Transformation Conversion : robotcorelib/Coordinate Transformation Conversion  InputRepresentation=Rotation Matrix  InputEulerSequence=ZYX  ShowTrVecInputPort=on  OutputRepresentation=Quaternion  OutputEulerSequence=ZYX  ShowTrVecOutputPort=on  SimulateUsing=Interpreted execution
  Inner-loop control : Subsystem
  Outer-loop control : MATLAB Function  TreatAsAtomicUnit=on
  Planner : Subsystem
  Quadrotor dynamics : Subsystem
  Scope{,1..5} (6 alike) : Scope
      Scope settings: ActiveDisplayYMinimum=-1.2E-5  ActiveDisplayYMaximum=1.2E-5
      Scope1 settings: ActiveDisplayYMinimum=-1.2E-5  ActiveDisplayYMaximum=1.2E-5
      Scope2 settings: ActiveDisplayYMinimum=-3.9E-5  ActiveDisplayYMaximum=1.1E-5  DataLoggingVariableName=ScopeData2
      Scope3 settings: ActiveDisplayYMinimum=-0.00022  ActiveDisplayYMaximum=0.00011  DataLoggingVariableName=ScopeData3
      Scope4 settings: ActiveDisplayYMinimum=11.66748  ActiveDisplayYMaximum=12.03695  DataLoggingVariableName=ScopeData4
      Scope5 settings: ActiveDisplayYMinimum=-0.02035  ActiveDisplayYMaximum=0.02036  DataLoggingVariableName=ScopeData5
  Terminator : Terminator
  Terminator3 : Terminator
  Unit Delay1 u0=12N : UnitDelay  InitialCondition=12  SampleTime=Ts
  Unit Delay2 : UnitDelay  InitialCondition=[0 0 0]  SampleTime=Ts
  Zero-Order Hold{1..5} (5 alike) : ZeroOrderHold  SampleTime=Ts
  Lin Acc : Outport
  Lin Vel : Outport  Port=2
  Lin Pos : Outport  Port=3
  Rotation : Outport  Port=4
  wires:
  Zero-Order Hold5/1 -> Lin Acc/1
  Quadrotor dynamics/7(lin_acc) -> Zero-Order Hold5/1
  Planner/1(position_des) -> Outer-loop control/4(position_des)
  Quadrotor dynamics/1(Position) -> Zero-Order Hold4/1
  Quadrotor dynamics/3(Rb) -> Zero-Order Hold2/1, Coordinate Transformation Conversion/1
  Quadrotor dynamics/4(dot_Rb) -> Terminator/1
  Planner/4(xb_des) -> Inner-loop control/4(xb_des)
  Inner-loop control/1(tau) -> Unit Delay2/1
  Planner/2(linear_velocity_des) -> Outer-loop control/5(vel_linear_des)
  Quadrotor dynamics/2(Linear_velocity) -> Zero-Order Hold1/1
  Quadrotor dynamics/6(dot_omega_bb) -> Terminator3/1
  Outer-loop control/3(err_p) -> Scope2/1
  Coordinate Transformation Conversion/1 -> Rotation/1
  Quadrotor dynamics/5(omega_bb) -> Zero-Order Hold3/1
  Zero-Order Hold2/1 -> Inner-loop control/2(Rb), Outer-loop control/3(Rb)
  References/1 -> Planner/1(References)
  Planner/3(linear_acceleration_des) -> Outer-loop control/6(acc_linear_des)
  Inner-loop control/3(err_W) -> Scope1/1
  Outer-loop control/2(zb_des) -> Inner-loop control/1(zb_des)
  Inner-loop control/2(err_R) -> Scope/1
  Outer-loop control/1(uT) -> Unit Delay1 u0=12N/1
  Unit Delay2/1 -> Quadrotor dynamics/2(tau_b), Scope5/1
  Zero-Order Hold3/1 -> Inner-loop control/3(omega_bb)
  Unit Delay1 u0=12N/1 -> Scope4/1, Quadrotor dynamics/1(uT)
  Outer-loop control/4(dot_err_p) -> Scope3/1
  Zero-Order Hold1/1 -> Outer-loop control/2(linear_vel), Lin Vel/1
  Zero-Order Hold4/1 -> Outer-loop control/1(position), Lin Pos/1

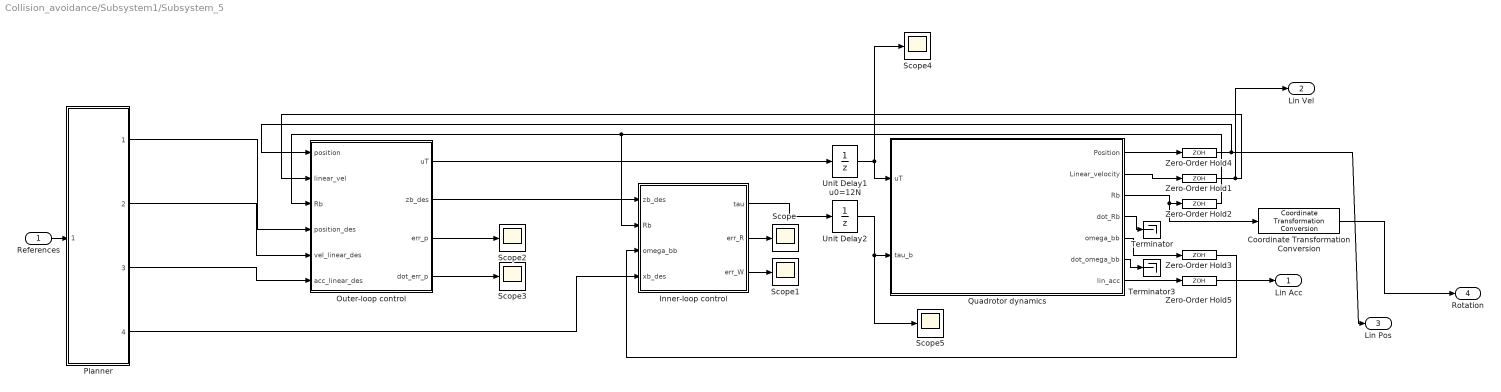
== system Collision_avoidance/Subsystem1/Subsystem_5 ==
  References : Inport
  Coordinate Transformation Conversion : robotcorelib/Coordinate Transformation Conversion  InputRepresentation=Rotation Matrix  InputEulerSequence=ZYX  ShowTrVecInputPort=on  OutputRepresentation=Quaternion  OutputEulerSequence=ZYX  ShowTrVecOutputPort=on  SimulateUsing=Interpreted execution
  Inner-loop control : Subsystem
  Outer-loop control : MATLAB Function  TreatAsAtomicUnit=on
  Planner : Subsystem
  Quadrotor dynamics : Subsystem
  Scope{,1..5} (6 alike) : Scope
      Scope settings: ActiveDisplayYMinimum=-1.2E-5  ActiveDisplayYMaximum=1.2E-5
      Scope1 settings: ActiveDisplayYMinimum=-1.2E-5  ActiveDisplayYMaximum=1.2E-5
      Scope2 settings: ActiveDisplayYMinimum=-3.9E-5  ActiveDisplayYMaximum=1.1E-5  DataLoggingVariableName=ScopeData2
      Scope3 settings: ActiveDisplayYMinimum=-0.00022  ActiveDisplayYMaximum=0.00011  DataLoggingVariableName=ScopeData3
      Scope4 settings: ActiveDisplayYMinimum=11.66748  ActiveDisplayYMaximum=12.03695  DataLoggingVariableName=ScopeData4
      Scope5 settings: ActiveDisplayYMinimum=-0.02035  ActiveDisplayYMaximum=0.02036  DataLoggingVariableName=ScopeData5
  Terminator : Terminator
  Terminator3 : Terminator
  Unit Delay1 u0=12N : UnitDelay  InitialCondition=12  SampleTime=Ts
  Unit Delay2 : UnitDelay  InitialCondition=[0 0 0]  SampleTime=Ts
  Zero-Order Hold{1..5} (5 alike) : ZeroOrderHold  SampleTime=Ts
  Lin Acc : Outport
  Lin Vel : Outport  Port=2
  Lin Pos : Outport  Port=3
  Rotation : Outport  Port=4
  wires:
  Zero-Order Hold5/1 -> Lin Acc/1
  Quadrotor dynamics/7(lin_acc) -> Zero-Order Hold5/1
  Planner/1(position_des) -> Outer-loop control/4(position_des)
  Quadrotor dynamics/1(Position) -> Zero-Order Hold4/1
  Quadrotor dynamics/3(Rb) -> Zero-Order Hold2/1, Coordinate Transformation Conversion/1
  Quadrotor dynamics/4(dot_Rb) -> Terminator/1
  Planner/4(xb_des) -> Inner-loop control/4(xb_des)
  Inner-loop control/1(tau) -> Unit Delay2/1
  Planner/2(linear_velocity_des) -> Outer-loop control/5(vel_linear_des)
  Quadrotor dynamics/2(Linear_velocity) -> Zero-Order Hold1/1
  Quadrotor dynamics/6(dot_omega_bb) -> Terminator3/1
  Outer-loop control/3(err_p) -> Scope2/1
  Coordinate Transformation Conversion/1 -> Rotation/1
  Quadrotor dynamics/5(omega_bb) -> Zero-Order Hold3/1
  Zero-Order Hold2/1 -> Inner-loop control/2(Rb), Outer-loop control/3(Rb)
  References/1 -> Planner/1(References)
  Planner/3(linear_acceleration_des) -> Outer-loop control/6(acc_linear_des)
  Inner-loop control/3(err_W) -> Scope1/1
  Outer-loop control/2(zb_des) -> Inner-loop control/1(zb_des)
  Inner-loop control/2(err_R) -> Scope/1
  Outer-loop control/1(uT) -> Unit Delay1 u0=12N/1
  Unit Delay2/1 -> Quadrotor dynamics/2(tau_b), Scope5/1
  Zero-Order Hold3/1 -> Inner-loop control/3(omega_bb)
  Unit Delay1 u0=12N/1 -> Scope4/1, Quadrotor dynamics/1(uT)
  Outer-loop control/4(dot_err_p) -> Scope3/1
  Zero-Order Hold1/1 -> Outer-loop control/2(linear_vel), Lin Vel/1
  Zero-Order Hold4/1 -> Outer-loop control/1(position), Lin Pos/1

== system Collision_avoidance/Subsystem1/Subsystem_1/Inner-loop control ==
  zb_des : Inport
  Rb : Inport  Port=2
  omega_bb : Inport  Port=3
  xb_des : Inport  Port=4
  Derivation : DiscreteTransferFcn  Numerator=[1 -1]  Denominator=[Ts 0]  InitialStates=[1 0 0;0 1 0;0 0 1]  SampleTime=Ts
  Derivation1 : DiscreteTransferFcn  Numerator=[1 -1]  Denominator=[Ts 0]  InitialStates=[0 0 0]  SampleTime=Ts
  Inner-loop control : MATLAB Function  TreatAsAtomicUnit=on
  Unit Delay1 : UnitDelay  InitialCondition=eye(3)  SampleTime=Ts
  Unit Delay3 : UnitDelay  InitialCondition=[0 0 0]  SampleTime=Ts
  tau : Outport
  err_R : Outport  Port=2
  err_W : Outport  Port=3
  wires:
  Inner-loop control/2(omega_bb_des) -> Derivation1/1
  Inner-loop control/1(Rb_des) -> Derivation/1
  omega_bb/1 -> Inner-loop control/4(omega_bb)
  zb_des/1 -> Inner-loop control/1(zb_des)
  Derivation/1 -> Unit Delay1/1
  Unit Delay3/1 -> Inner-loop control/5(dot_omega_bb_des)
  Inner-loop control/5(err_W) -> err_W/1
  Derivation1/1 -> Unit Delay3/1
  Unit Delay1/1 -> Inner-loop control/3(dot_Rb_des)
  Inner-loop control/3(tau) -> tau/1
  Rb/1 -> Inner-loop control/2(Rb)
  Inner-loop control/4(err_R) -> err_R/1
  xb_des/1 -> Inner-loop control/6(xb_des)

== system Collision_avoidance/Subsystem1/Subsystem_1/Planner ==
  References : Inport
  Constant : Constant  Value=0
  Demux : Demux  Outputs=10
  Mux{1..4} (4 alike) : Mux  Inputs=3
  Trigonometric Function : Trigonometry
  Trigonometric Function1 : Trigonometry  Operator=cos
  position_des : Outport
  linear_velocity_des : Outport  Port=2
  linear_acceleration_des : Outport  Port=3
  xb_des : Outport  Port=4
  wires:
  References/1 -> Demux/1
  Demux/10 -> Trigonometric Function1/1, Trigonometric Function/1
  Demux/9 -> Mux1/3
  Demux/8 -> Mux1/2
  Demux/7 -> Mux1/1
  Demux/6 -> Mux3/3
  Demux/5 -> Mux3/2
  Demux/4 -> Mux3/1
  Demux/3 -> Mux2/3
  Demux/2 -> Mux2/2
  Demux/1 -> Mux2/1
  Constant/1 -> Mux4/3
  Trigonometric Function1/1 -> Mux4/1
  Trigonometric Function/1 -> Mux4/2
  Mux4/1 -> xb_des/1
  Mux2/1 -> position_des/1
  Mux3/1 -> linear_velocity_des/1
  Mux1/1 -> linear_acceleration_des/1

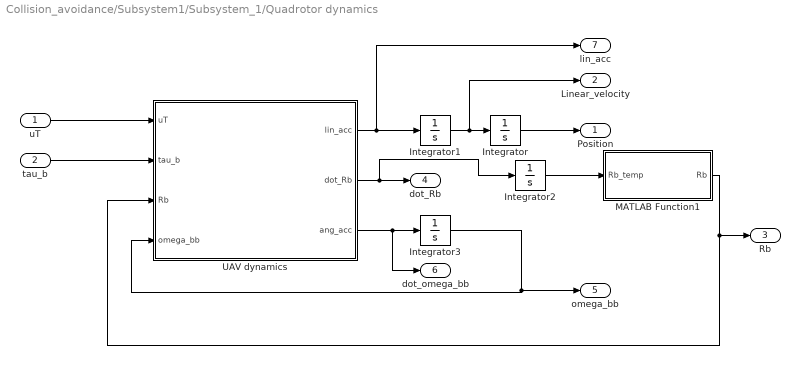
== system Collision_avoidance/Subsystem1/Subsystem_1/Quadrotor dynamics ==
  uT : Inport
  tau_b : Inport  Port=2
  Integrator : Integrator  InitialCondition=init_0
  Integrator1 : Integrator  InitialCondition=lin_vel_0
  Integrator2 : Integrator  InitialCondition=[1 0 0; 0 1 0;0 0 1]
  Integrator3 : Integrator  InitialCondition=w_bb_0
  MATLAB Function1 : MATLAB Function  TreatAsAtomicUnit=on
  UAV dynamics : MATLAB Function  TreatAsAtomicUnit=on
  Position : Outport
  Linear_velocity : Outport  Port=2
  Rb : Outport  Port=3
  dot_Rb : Outport  Port=4
  omega_bb : Outport  Port=5
  dot_omega_bb : Outport  Port=6
  lin_acc : Outport  Port=7
  wires:
  Integrator2/1 -> MATLAB Function1/1(Rb_temp)
  MATLAB Function1/1(Rb) -> UAV dynamics/3(Rb), Rb/1
  UAV dynamics/2(dot_Rb) -> dot_Rb/1, Integrator2/1
  Integrator3/1 -> omega_bb/1, UAV dynamics/4(omega_bb)
  Integrator1/1 -> Integrator/1, Linear_velocity/1
  uT/1 -> UAV dynamics/1(uT)
  UAV dynamics/1(lin_acc) -> Integrator1/1, lin_acc/1
  UAV dynamics/3(ang_acc) -> Integrator3/1, dot_omega_bb/1
  Integrator/1 -> Position/1
  tau_b/1 -> UAV dynamics/2(tau_b)

== system Collision_avoidance/Subsystem1/Subsystem_2/Inner-loop control ==
  zb_des : Inport
  Rb : Inport  Port=2
  omega_bb : Inport  Port=3
  xb_des : Inport  Port=4
  Derivation : DiscreteTransferFcn  Numerator=[1 -1]  Denominator=[Ts 0]  InitialStates=[1 0 0;0 1 0;0 0 1]  SampleTime=Ts
  Derivation1 : DiscreteTransferFcn  Numerator=[1 -1]  Denominator=[Ts 0]  InitialStates=[0 0 0]  SampleTime=Ts
  Inner-loop control : MATLAB Function  TreatAsAtomicUnit=on
  Unit Delay1 : UnitDelay  InitialCondition=eye(3)  SampleTime=Ts
  Unit Delay3 : UnitDelay  InitialCondition=[0 0 0]  SampleTime=Ts
  tau : Outport
  err_R : Outport  Port=2
  err_W : Outport  Port=3
  wires:
  Inner-loop control/2(omega_bb_des) -> Derivation1/1
  Inner-loop control/1(Rb_des) -> Derivation/1
  omega_bb/1 -> Inner-loop control/4(omega_bb)
  zb_des/1 -> Inner-loop control/1(zb_des)
  Derivation/1 -> Unit Delay1/1
  Unit Delay3/1 -> Inner-loop control/5(dot_omega_bb_des)
  Inner-loop control/5(err_W) -> err_W/1
  Derivation1/1 -> Unit Delay3/1
  Unit Delay1/1 -> Inner-loop control/3(dot_Rb_des)
  Inner-loop control/3(tau) -> tau/1
  Rb/1 -> Inner-loop control/2(Rb)
  Inner-loop control/4(err_R) -> err_R/1
  xb_des/1 -> Inner-loop control/6(xb_des)

== system Collision_avoidance/Subsystem1/Subsystem_2/Planner ==
  References : Inport
  Constant : Constant  Value=0
  Demux : Demux  Outputs=10
  Mux{1..4} (4 alike) : Mux  Inputs=3
  Trigonometric Function : Trigonometry
  Trigonometric Function1 : Trigonometry  Operator=cos
  position_des : Outport
  linear_velocity_des : Outport  Port=2
  linear_acceleration_des : Outport  Port=3
  xb_des : Outport  Port=4
  wires:
  References/1 -> Demux/1
  Demux/10 -> Trigonometric Function1/1, Trigonometric Function/1
  Demux/9 -> Mux1/3
  Demux/8 -> Mux1/2
  Demux/7 -> Mux1/1
  Demux/6 -> Mux3/3
  Demux/5 -> Mux3/2
  Demux/4 -> Mux3/1
  Demux/3 -> Mux2/3
  Demux/2 -> Mux2/2
  Demux/1 -> Mux2/1
  Constant/1 -> Mux4/3
  Trigonometric Function1/1 -> Mux4/1
  Trigonometric Function/1 -> Mux4/2
  Mux4/1 -> xb_des/1
  Mux2/1 -> position_des/1
  Mux3/1 -> linear_velocity_des/1
  Mux1/1 -> linear_acceleration_des/1

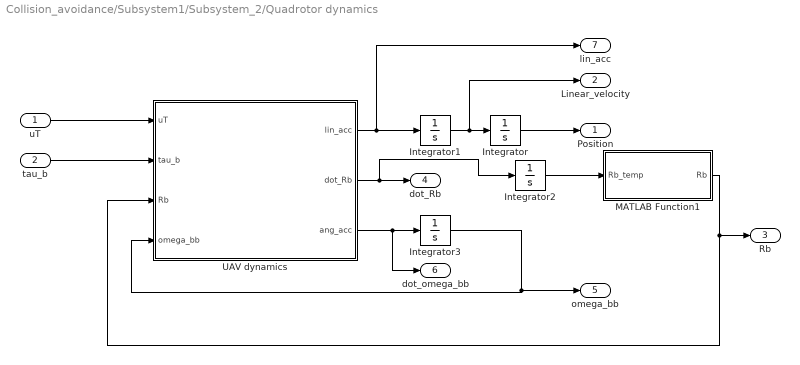
== system Collision_avoidance/Subsystem1/Subsystem_2/Quadrotor dynamics ==
  uT : Inport
  tau_b : Inport  Port=2
  Integrator : Integrator  InitialCondition=init_1
  Integrator1 : Integrator  InitialCondition=lin_vel_0
  Integrator2 : Integrator  InitialCondition=[1 0 0; 0 1 0;0 0 1]
  Integrator3 : Integrator  InitialCondition=w_bb_0
  MATLAB Function1 : MATLAB Function  TreatAsAtomicUnit=on
  UAV dynamics : MATLAB Function  TreatAsAtomicUnit=on
  Position : Outport
  Linear_velocity : Outport  Port=2
  Rb : Outport  Port=3
  dot_Rb : Outport  Port=4
  omega_bb : Outport  Port=5
  dot_omega_bb : Outport  Port=6
  lin_acc : Outport  Port=7
  wires:
  Integrator2/1 -> MATLAB Function1/1(Rb_temp)
  MATLAB Function1/1(Rb) -> UAV dynamics/3(Rb), Rb/1
  UAV dynamics/2(dot_Rb) -> dot_Rb/1, Integrator2/1
  Integrator3/1 -> omega_bb/1, UAV dynamics/4(omega_bb)
  Integrator1/1 -> Integrator/1, Linear_velocity/1
  uT/1 -> UAV dynamics/1(uT)
  UAV dynamics/1(lin_acc) -> Integrator1/1, lin_acc/1
  UAV dynamics/3(ang_acc) -> Integrator3/1, dot_omega_bb/1
  Integrator/1 -> Position/1
  tau_b/1 -> UAV dynamics/2(tau_b)

== system Collision_avoidance/Subsystem1/Subsystem_3/Inner-loop control ==
  zb_des : Inport
  Rb : Inport  Port=2
  omega_bb : Inport  Port=3
  xb_des : Inport  Port=4
  Derivation : DiscreteTransferFcn  Numerator=[1 -1]  Denominator=[Ts 0]  InitialStates=[1 0 0;0 1 0;0 0 1]  SampleTime=Ts
  Derivation1 : DiscreteTransferFcn  Numerator=[1 -1]  Denominator=[Ts 0]  InitialStates=[0 0 0]  SampleTime=Ts
  Inner-loop control : MATLAB Function  TreatAsAtomicUnit=on
  Unit Delay1 : UnitDelay  InitialCondition=eye(3)  SampleTime=Ts
  Unit Delay3 : UnitDelay  InitialCondition=[0 0 0]  SampleTime=Ts
  tau : Outport
  err_R : Outport  Port=2
  err_W : Outport  Port=3
  wires:
  Inner-loop control/2(omega_bb_des) -> Derivation1/1
  Inner-loop control/1(Rb_des) -> Derivation/1
  omega_bb/1 -> Inner-loop control/4(omega_bb)
  zb_des/1 -> Inner-loop control/1(zb_des)
  Derivation/1 -> Unit Delay1/1
  Unit Delay3/1 -> Inner-loop control/5(dot_omega_bb_des)
  Inner-loop control/5(err_W) -> err_W/1
  Derivation1/1 -> Unit Delay3/1
  Unit Delay1/1 -> Inner-loop control/3(dot_Rb_des)
  Inner-loop control/3(tau) -> tau/1
  Rb/1 -> Inner-loop control/2(Rb)
  Inner-loop control/4(err_R) -> err_R/1
  xb_des/1 -> Inner-loop control/6(xb_des)

== system Collision_avoidance/Subsystem1/Subsystem_3/Planner ==
  References : Inport
  Constant : Constant  Value=0
  Demux : Demux  Outputs=10
  Mux{1..4} (4 alike) : Mux  Inputs=3
  Trigonometric Function : Trigonometry
  Trigonometric Function1 : Trigonometry  Operator=cos
  position_des : Outport
  linear_velocity_des : Outport  Port=2
  linear_acceleration_des : Outport  Port=3
  xb_des : Outport  Port=4
  wires:
  References/1 -> Demux/1
  Demux/10 -> Trigonometric Function1/1, Trigonometric Function/1
  Demux/9 -> Mux1/3
  Demux/8 -> Mux1/2
  Demux/7 -> Mux1/1
  Demux/6 -> Mux3/3
  Demux/5 -> Mux3/2
  Demux/4 -> Mux3/1
  Demux/3 -> Mux2/3
  Demux/2 -> Mux2/2
  Demux/1 -> Mux2/1
  Constant/1 -> Mux4/3
  Trigonometric Function1/1 -> Mux4/1
  Trigonometric Function/1 -> Mux4/2
  Mux4/1 -> xb_des/1
  Mux2/1 -> position_des/1
  Mux3/1 -> linear_velocity_des/1
  Mux1/1 -> linear_acceleration_des/1

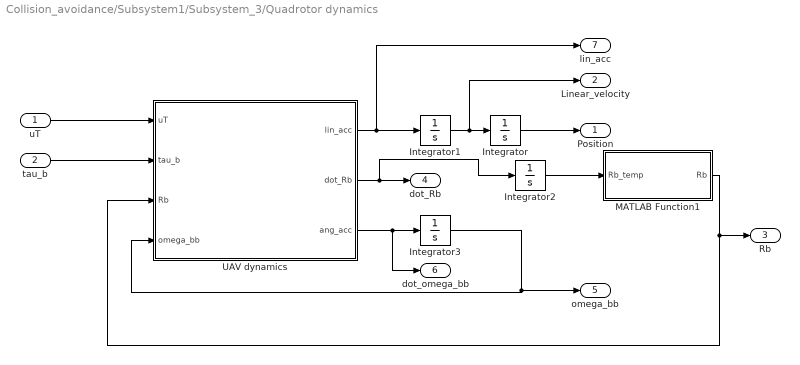
== system Collision_avoidance/Subsystem1/Subsystem_3/Quadrotor dynamics ==
  uT : Inport
  tau_b : Inport  Port=2
  Integrator : Integrator  InitialCondition=init_2
  Integrator1 : Integrator  InitialCondition=lin_vel_0
  Integrator2 : Integrator  InitialCondition=[1 0 0; 0 1 0;0 0 1]
  Integrator3 : Integrator  InitialCondition=w_bb_0
  MATLAB Function1 : MATLAB Function  TreatAsAtomicUnit=on
  UAV dynamics : MATLAB Function  TreatAsAtomicUnit=on
  Position : Outport
  Linear_velocity : Outport  Port=2
  Rb : Outport  Port=3
  dot_Rb : Outport  Port=4
  omega_bb : Outport  Port=5
  dot_omega_bb : Outport  Port=6
  lin_acc : Outport  Port=7
  wires:
  Integrator2/1 -> MATLAB Function1/1(Rb_temp)
  MATLAB Function1/1(Rb) -> UAV dynamics/3(Rb), Rb/1
  UAV dynamics/2(dot_Rb) -> dot_Rb/1, Integrator2/1
  Integrator3/1 -> omega_bb/1, UAV dynamics/4(omega_bb)
  Integrator1/1 -> Integrator/1, Linear_velocity/1
  uT/1 -> UAV dynamics/1(uT)
  UAV dynamics/1(lin_acc) -> Integrator1/1, lin_acc/1
  UAV dynamics/3(ang_acc) -> Integrator3/1, dot_omega_bb/1
  Integrator/1 -> Position/1
  tau_b/1 -> UAV dynamics/2(tau_b)

== system Collision_avoidance/Subsystem1/Subsystem_4/Inner-loop control ==
  zb_des : Inport
  Rb : Inport  Port=2
  omega_bb : Inport  Port=3
  xb_des : Inport  Port=4
  Derivation : DiscreteTransferFcn  Numerator=[1 -1]  Denominator=[Ts 0]  InitialStates=[1 0 0;0 1 0;0 0 1]  SampleTime=Ts
  Derivation1 : DiscreteTransferFcn  Numerator=[1 -1]  Denominator=[Ts 0]  InitialStates=[0 0 0]  SampleTime=Ts
  Inner-loop control : MATLAB Function  TreatAsAtomicUnit=on
  Unit Delay1 : UnitDelay  InitialCondition=eye(3)  SampleTime=Ts
  Unit Delay3 : UnitDelay  InitialCondition=[0 0 0]  SampleTime=Ts
  tau : Outport
  err_R : Outport  Port=2
  err_W : Outport  Port=3
  wires:
  Inner-loop control/2(omega_bb_des) -> Derivation1/1
  Inner-loop control/1(Rb_des) -> Derivation/1
  omega_bb/1 -> Inner-loop control/4(omega_bb)
  zb_des/1 -> Inner-loop control/1(zb_des)
  Derivation/1 -> Unit Delay1/1
  Unit Delay3/1 -> Inner-loop control/5(dot_omega_bb_des)
  Inner-loop control/5(err_W) -> err_W/1
  Derivation1/1 -> Unit Delay3/1
  Unit Delay1/1 -> Inner-loop control/3(dot_Rb_des)
  Inner-loop control/3(tau) -> tau/1
  Rb/1 -> Inner-loop control/2(Rb)
  Inner-loop control/4(err_R) -> err_R/1
  xb_des/1 -> Inner-loop control/6(xb_des)

== system Collision_avoidance/Subsystem1/Subsystem_4/Planner ==
  References : Inport
  Constant : Constant  Value=0
  Demux : Demux  Outputs=10
  Mux{1..4} (4 alike) : Mux  Inputs=3
  Trigonometric Function : Trigonometry
  Trigonometric Function1 : Trigonometry  Operator=cos
  position_des : Outport
  linear_velocity_des : Outport  Port=2
  linear_acceleration_des : Outport  Port=3
  xb_des : Outport  Port=4
  wires:
  References/1 -> Demux/1
  Demux/10 -> Trigonometric Function1/1, Trigonometric Function/1
  Demux/9 -> Mux1/3
  Demux/8 -> Mux1/2
  Demux/7 -> Mux1/1
  Demux/6 -> Mux3/3
  Demux/5 -> Mux3/2
  Demux/4 -> Mux3/1
  Demux/3 -> Mux2/3
  Demux/2 -> Mux2/2
  Demux/1 -> Mux2/1
  Constant/1 -> Mux4/3
  Trigonometric Function1/1 -> Mux4/1
  Trigonometric Function/1 -> Mux4/2
  Mux4/1 -> xb_des/1
  Mux2/1 -> position_des/1
  Mux1/1 -> linear_acceleration_des/1
  Mux3/1 -> linear_velocity_des/1

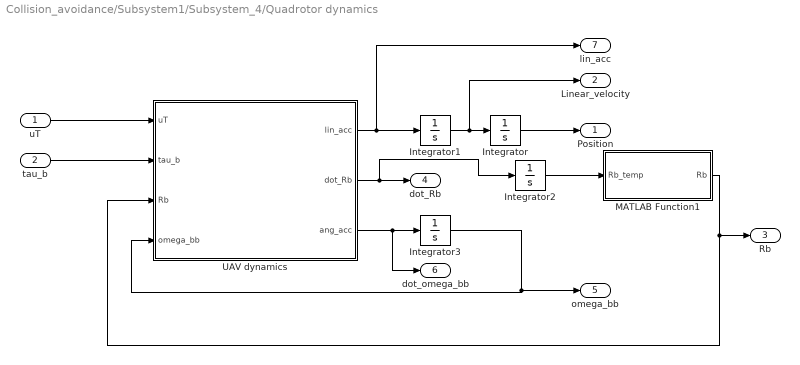
== system Collision_avoidance/Subsystem1/Subsystem_4/Quadrotor dynamics ==
  uT : Inport
  tau_b : Inport  Port=2
  Integrator : Integrator  InitialCondition=init_3
  Integrator1 : Integrator  InitialCondition=lin_vel_0
  Integrator2 : Integrator  InitialCondition=[1 0 0; 0 1 0;0 0 1]
  Integrator3 : Integrator  InitialCondition=w_bb_0
  MATLAB Function1 : MATLAB Function  TreatAsAtomicUnit=on
  UAV dynamics : MATLAB Function  TreatAsAtomicUnit=on
  Position : Outport
  Linear_velocity : Outport  Port=2
  Rb : Outport  Port=3
  dot_Rb : Outport  Port=4
  omega_bb : Outport  Port=5
  dot_omega_bb : Outport  Port=6
  lin_acc : Outport  Port=7
  wires:
  Integrator2/1 -> MATLAB Function1/1(Rb_temp)
  MATLAB Function1/1(Rb) -> UAV dynamics/3(Rb), Rb/1
  UAV dynamics/2(dot_Rb) -> dot_Rb/1, Integrator2/1
  Integrator3/1 -> omega_bb/1, UAV dynamics/4(omega_bb)
  Integrator1/1 -> Integrator/1, Linear_velocity/1
  uT/1 -> UAV dynamics/1(uT)
  UAV dynamics/1(lin_acc) -> Integrator1/1, lin_acc/1
  UAV dynamics/3(ang_acc) -> Integrator3/1, dot_omega_bb/1
  Integrator/1 -> Position/1
  tau_b/1 -> UAV dynamics/2(tau_b)

== system Collision_avoidance/Subsystem1/Subsystem_5/Inner-loop control ==
  zb_des : Inport
  Rb : Inport  Port=2
  omega_bb : Inport  Port=3
  xb_des : Inport  Port=4
  Derivation : DiscreteTransferFcn  Numerator=[1 -1]  Denominator=[Ts 0]  InitialStates=[1 0 0;0 1 0;0 0 1]  SampleTime=Ts
  Derivation1 : DiscreteTransferFcn  Numerator=[1 -1]  Denominator=[Ts 0]  InitialStates=[0 0 0]  SampleTime=Ts
  Inner-loop control : MATLAB Function  TreatAsAtomicUnit=on
  Unit Delay1 : UnitDelay  InitialCondition=eye(3)  SampleTime=Ts
  Unit Delay3 : UnitDelay  InitialCondition=[0 0 0]  SampleTime=Ts
  tau : Outport
  err_R : Outport  Port=2
  err_W : Outport  Port=3
  wires:
  Inner-loop control/2(omega_bb_des) -> Derivation1/1
  Inner-loop control/1(Rb_des) -> Derivation/1
  omega_bb/1 -> Inner-loop control/4(omega_bb)
  zb_des/1 -> Inner-loop control/1(zb_des)
  Derivation/1 -> Unit Delay1/1
  Unit Delay3/1 -> Inner-loop control/5(dot_omega_bb_des)
  Inner-loop control/5(err_W) -> err_W/1
  Derivation1/1 -> Unit Delay3/1
  Unit Delay1/1 -> Inner-loop control/3(dot_Rb_des)
  Inner-loop control/3(tau) -> tau/1
  Rb/1 -> Inner-loop control/2(Rb)
  Inner-loop control/4(err_R) -> err_R/1
  xb_des/1 -> Inner-loop control/6(xb_des)

== system Collision_avoidance/Subsystem1/Subsystem_5/Planner ==
  References : Inport
  Constant : Constant  Value=0
  Demux : Demux  Outputs=10
  Mux{1..4} (4 alike) : Mux  Inputs=3
  Trigonometric Function : Trigonometry
  Trigonometric Function1 : Trigonometry  Operator=cos
  position_des : Outport
  linear_velocity_des : Outport  Port=2
  linear_acceleration_des : Outport  Port=3
  xb_des : Outport  Port=4
  wires:
  References/1 -> Demux/1
  Demux/10 -> Trigonometric Function1/1, Trigonometric Function/1
  Demux/9 -> Mux1/3
  Demux/8 -> Mux1/2
  Demux/7 -> Mux1/1
  Demux/6 -> Mux3/3
  Demux/5 -> Mux3/2
  Demux/4 -> Mux3/1
  Demux/3 -> Mux2/3
  Demux/2 -> Mux2/2
  Demux/1 -> Mux2/1
  Constant/1 -> Mux4/3
  Trigonometric Function1/1 -> Mux4/1
  Trigonometric Function/1 -> Mux4/2
  Mux4/1 -> xb_des/1
  Mux2/1 -> position_des/1
  Mux1/1 -> linear_acceleration_des/1
  Mux3/1 -> linear_velocity_des/1
